simulink model "lab4"  (R2026a)
settings: Solver=VariableStepAuto  StopTime=30
values from neighbouring files (symbols this model uses):
  A = [0,              0,             w0,        0 ... (first row only)    [lab3_t3.m]    (also in lab4_m.m = [          0,            0,      omega0,           0)
  B = [0 ... (first row only)    [lab4_m.m]
  Bd = [0 ... (first row only)    [lab4_m.m]
  K = place(A, B_I, desired_poles)    [lab3_t3.m]    (also in lab4_m.m = K_1_2)
  K_1_2 = place(A, B, poles_1_2)    [lab4_m.m]
  K_i_reg = K_aug_all(1:4)    [lab4_m.m]
  Ki = -K_aug_all(5)    [lab4_m.m]
  kr = 1 / (-C * inv(A - B*K) * B)    [lab4_m.m]
  L_slow = place(A', C', poles_obs_slow)'    [lab4_m.m]
libraries: simulink x3

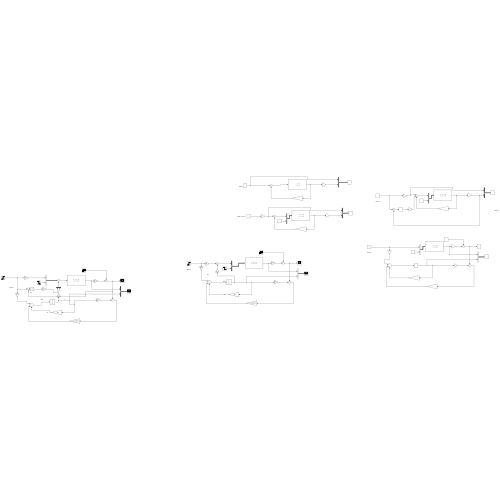
[thumbnail: Simulink's stored preview of the top-level diagram]
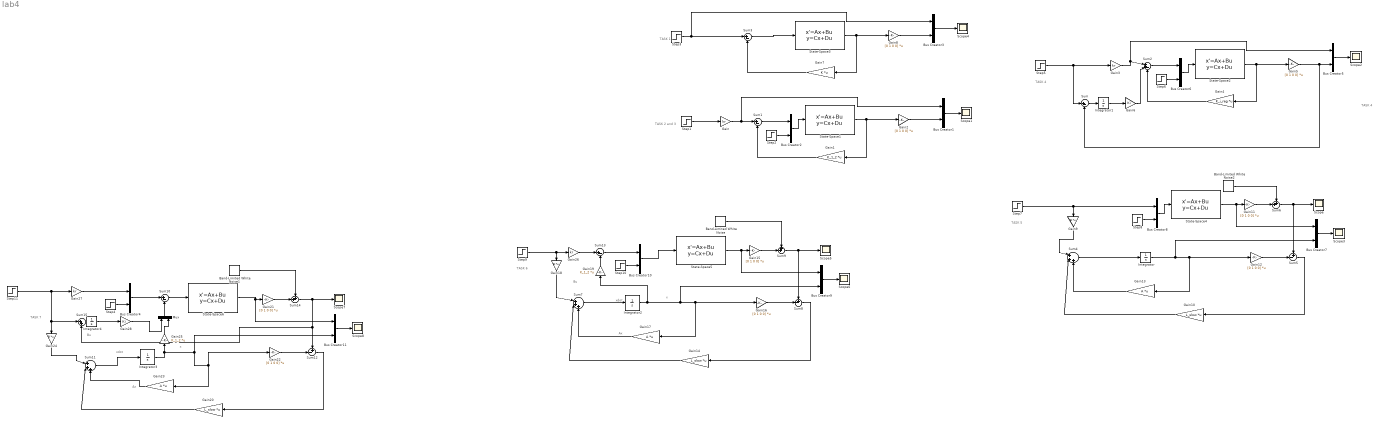
== system lab4 ==
  note: Bu
  note: Ax
  note: x
  note: xdot
  note: TASK 1
  note: TASK 2 and 3
  note: TASK 4
  note: TASK 4
  note: TASK 5
  note: TASK 6
  note: TASK 7
  note: xdot
  note: x
  note: Bu
  note: Ax
  Band-Limited White Noise : simulink/Sources/Band-Limited White Noise  Cov=[0.0005]  Ts=0.1  seed=[23341]
  Band-Limited White Noise1 : simulink/Sources/Band-Limited White Noise  Cov=[0.0005]  Ts=0.1  seed=[23341]
  Band-Limited White Noise2 : simulink/Sources/Band-Limited White Noise  Cov=[0.0005]  Ts=0.1  seed=[23341]
  Bus Creator{1..11} (11 alike) : BusCreator  Inputs=2
  Gain{,3,26..27} (4 alike) : Gain  Gain=kr
  Gain1 : Gain  Gain=K_1_2  Multiplication=Matrix(K*u)
  Gain10 : Gain  Gain=L_slow  Multiplication=Matrix(K*u)
  Gain{2,5,8,11..12,15..16,21..22} (9 alike) : Gain  Gain=[0 1 0 0]  Multiplication=Matrix(K*u)
  Gain13 : Gain  Gain=A  Multiplication=Matrix(K*u)
  Gain14 : Gain  Gain=L_slow  Multiplication=Matrix(K*u)
  Gain17 : Gain  Gain=A  Multiplication=Matrix(K*u)
  Gain18 : Gain  Gain=B  Multiplication=Matrix(K*u)
  Gain19 : Gain  Gain=K_1_2  Multiplication=Matrix(K*u)
  Gain20 : Gain  Gain=L_slow  Multiplication=Matrix(K*u)
  Gain23 : Gain  Gain=A  Multiplication=Matrix(K*u)
  Gain24 : Gain  Gain=B  Multiplication=Matrix(K*u)
  Gain25 : Gain  Gain=K_1_2  Multiplication=Matrix(K*u)
  Gain28 : Gain  Gain=Ki
  Gain4 : Gain  Gain=K_i_reg  Multiplication=Matrix(K*u)
  Gain6 : Gain  Gain=Ki
  Gain7 : Gain  Gain=K  Multiplication=Matrix(K*u)
  Gain9 : Gain  Gain=B  Multiplication=Matrix(K*u)
  Integrator{,1..4} (5 alike) : Integrator
  Mux : Mux  Inputs=2
  Scope{,1..8} (9 alike) : Scope
      Scope settings: ActiveDisplayYMinimum=-2.6335028187661971  ActiveDisplayYMaximum=22.20466826951543  DataLoggingVariableName=ScopeData4
      Scope1 settings: ActiveDisplayYMinimum=-2.3833333333353988  ActiveDisplayYMaximum=21.450000000018594
      Scope2 settings: ActiveDisplayYMinimum=-2.3833333333353988  ActiveDisplayYMaximum=21.450000000018594  DataLoggingVariableName=ScopeData2
      Scope3 settings: ActiveDisplayYMinimum=-15.894708744203601  ActiveDisplayYMaximum=33.905632916389834  DataLoggingVariableName=ScopeData3
      Scope4 settings: ActiveDisplayYMinimum=-0.32827814261350396  ActiveDisplayYMaximum=0.51777105992235473
      Scope5 settings: ActiveDisplayYMinimum=-1.0275328267117055E+11  ActiveDisplayYMaximum=1.0737645995939032E+11  DataLoggingVariableName=ScopeData5
      Scope6 settings: ActiveDisplayYMinimum=-5.4423832466964326E+12  ActiveDisplayYMaximum=7.8702656903246934E+12  DataLoggingVariableName=ScopeData6
      Scope7 settings: ActiveDisplayYMinimum=-5.9753049160396826E+8  ActiveDisplayYMaximum=8.078710650567534E+8  DataLoggingVariableName=ScopeData7
      Scope8 settings: ActiveDisplayYMinimum=-3.4543187159854383E+35  ActiveDisplayYMaximum=2.4551274984006983E+36  DataLoggingVariableName=ScopeData8
  State-Space{1..2,4..6} (5 alike) : StateSpace  A=A  B=[B Bd]  C=eye(4)  D=[0 0; 0 0; 0 0;0 0 ]  InitialCondition=0
  State-Space3 : StateSpace  A=A  B=B  C=eye(4)  D=zeros(4,1)  InitialCondition=0
  Step{1,3,5,7,9,11} (6 alike) : Step  SampleTime=0
  Step{4,6,8,10} (4 alike) : Step  Time=10  FinalValue=-1  SampleTime=0
  Step2 : Step  Time=10  FinalValue=0  SampleTime=0
  Sum{,1,3,10,13} (5 alike) : Sum  Inputs=|+-
  Sum11 : Sum  Inputs=|+++
  Sum12 : Sum  Inputs=+-|
  Sum14 : Sum  Inputs=++|
  Sum15 : Sum  Inputs=|++
  Sum2 : Sum  Inputs=|++-
  Sum4 : Sum  Inputs=|+++
  Sum5 : Sum  Inputs=+-|
  Sum6 : Sum  Inputs=++|
  Sum7 : Sum  Inputs=|+++
  Sum8 : Sum  Inputs=+-|
  Sum9 : Sum  Inputs=++|
  wires:
  Step3/1 -> Sum3/1, Bus Creator3/1
  Bus Creator3/1 -> Scope4/1
  Gain7/1 -> Sum3/2
  Gain8/1 -> Bus Creator3/2
  Sum3/1 -> State-Space3/1
  State-Space3/1 -> Gain7/1, Gain8/1
  Step1/1 -> Gain/1
  Bus Creator2/1 -> State-Space1/1
  Step2/1 -> Bus Creator2/2
  Gain2/1 -> Bus Creator1/2
  Bus Creator1/1 -> Scope1/1
  State-Space1/1 -> Gain1/1, Gain2/1
  Sum1/1 -> Bus Creator2/1
  Gain1/1 -> Sum1/2
  Gain/1 -> Sum1/1, Bus Creator1/1
  Bus Creator6/1 -> State-Space2/1
  Step6/1 -> Bus Creator6/2
  State-Space2/1 -> Gain4/1, Gain5/1
  Gain4/1 -> Sum2/3
  Sum2/1 -> Bus Creator6/1
  Gain3/1 -> Bus Creator5/1, Sum2/1
  Step5/1 -> Gain3/1, Sum/1
  Bus Creator5/1 -> Scope2/1
  Sum/1 -> Integrator1/1
  Integrator1/1 -> Gain6/1
  Gain6/1 -> Sum2/2
  Gain5/1 -> Sum/2, Bus Creator5/2
  Bus Creator8/1 -> State-Space4/1
  Step7/1 -> Gain9/1, Bus Creator8/1
  State-Space4/1 -> Bus Creator7/1, Gain11/1
  Step8/1 -> Bus Creator8/2
  Bus Creator7/1 -> Scope3/1
  Gain9/1 -> Sum4/1
  Sum4/1 -> Integrator/1
  Gain12/1 -> Sum5/2
  Sum5/1 -> Gain10/1
  Gain13/1 -> Sum4/3
  Gain10/1 -> Sum4/2
  Integrator/1 -> Bus Creator7/2, Gain13/1, Gain12/1
  Gain11/1 -> Sum6/2
  Sum6/1 -> Scope/1, Sum5/1
  Band-Limited White Noise2/1 -> Sum6/1
  Band-Limited White Noise/1 -> Sum9/1
  Gain15/1 -> Sum9/2
  Gain16/1 -> Sum8/2
  Sum9/1 -> Scope5/1, Sum8/1
  Gain17/1 -> Sum7/3
  Integrator2/1 -> Bus Creator9/2, Gain17/1, Gain16/1, Gain19/1
  Sum7/1 -> Integrator2/1
  Sum8/1 -> Gain14/1
  Gain18/1 -> Sum7/1
  Bus Creator9/1 -> Scope6/1
  Step10/1 -> Bus Creator10/2
  State-Space5/1 -> Bus Creator9/1, Gain15/1
  Gain14/1 -> Sum7/2
  Gain19/1 -> Sum13/2
  Sum13/1 -> Bus Creator10/1
  Bus Creator10/1 -> State-Space5/1
  Sum11/1 -> Integrator3/1
  Sum12/1 -> Gain20/1
  Band-Limited White Noise1/1 -> Sum14/1
  Gain21/1 -> Sum14/2
  State-Space6/1 -> Bus Creator11/1, Gain21/1
  Bus Creator4/1 -> Sum10/1
  Gain22/1 -> Sum12/2
  Gain20/1 -> Sum11/2
  Integrator3/1 -> Bus Creator11/2, Gain22/1, Gain23/1, Gain25/1
  Gain27/1 -> Bus Creator4/1
  Gain23/1 -> Sum11/3
  Gain24/1 -> Sum11/1
  Step4/1 -> Bus Creator4/2
  Bus Creator11/1 -> Scope8/1
  Sum14/1 -> Scope7/1, Sum15/2, Sum12/1
  Gain25/1 -> Mux/2
  Step9/1 -> Gain26/1, Gain18/1
  Step11/1 -> Gain27/1, Sum15/1, Gain24/1
  Sum15/1 -> Integrator4/1
  Integrator4/1 -> Gain28/1
  Gain28/1 -> Mux/1
  Mux/1 -> Sum10/2
  Sum10/1 -> State-Space6/1
  Gain26/1 -> Sum13/1
